simulink model "Lab3_2_4_5"  (R2024b)
settings: Solver=VariableStepAuto  StartTime=0.0  StopTime=10.0  RelTol=1e-3
undefined symbols (not defined in the file): A, B, D, K, KI, Nr
libraries: simulink_extras x2
settings Model: Creator=vahid  LastModifiedBy=vahid

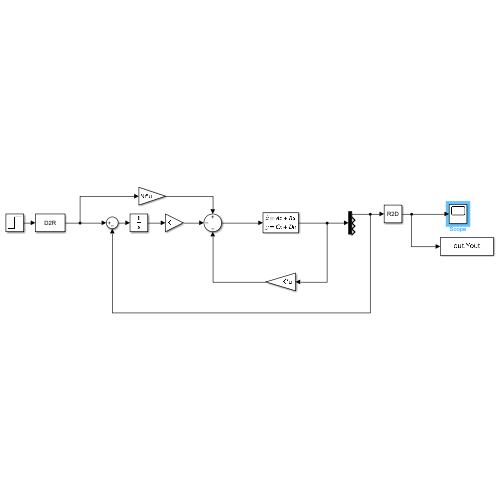
[thumbnail: Simulink's stored preview of the top-level diagram]
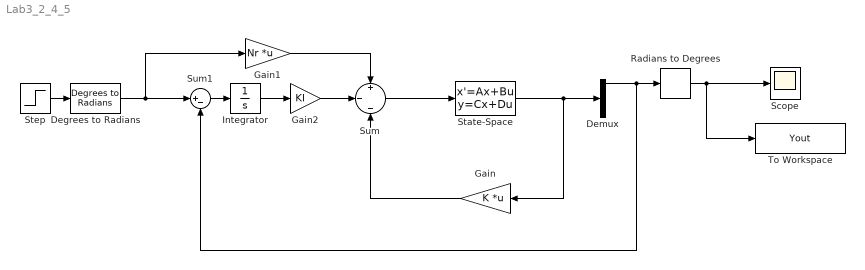
== system Lab3_2_4_5 ==
  Degrees to Radians : simulink_extras/Transformations/Degrees to Radians
  Demux : Demux
  Gain : Gain  Gain=K  Multiplication=Matrix(K*u)
  Gain1 : Gain  Gain=Nr  Multiplication=Matrix(K*u)
  Gain2 : Gain  Gain=KI
  Integrator : Integrator
  Radians to Degrees : simulink_extras/Transformations/Radians to Degrees
  Scope : Scope
  State-Space : StateSpace  A=A  B=B  C=eye(4)  D=D  InitialCondition=0
  Step : Step  Time=0  After=50  SampleTime=0
  Sum : Sum  Inputs=+|-|-
  Sum1 : Sum  Inputs=|+-
  To Workspace : ToWorkspace  VariableName=Yout  SaveFormat=Timeseries  SampleTime=-1
  wires:
  Gain2/1 -> Sum/2
  Gain/1 -> Sum/3
  Demux/1 -> Sum1/2, Radians to Degrees/1
  Radians to Degrees/1 -> To Workspace/1, Scope/1
  Step/1 -> Degrees to Radians/1
  Gain1/1 -> Sum/1
  Sum1/1 -> Integrator/1
  Sum/1 -> State-Space/1
  Degrees to Radians/1 -> Gain1/1, Sum1/1
  State-Space/1 -> Demux/1, Gain/1
  Integrator/1 -> Gain2/1
